simulink model "W06_8_ned"  (R2024b)
settings: Solver=ode4  StartTime=0  StopTime=120  FixedStep=h  RelTol=1e-3
InitFcn:
  | addpath(fullfile(fileparts(fileparts(fileparts(get_param(bdroot, 'FileName')))), '_tools'), fileparts(get_param(bdroot, 'FileName'))); run_alone('W06', bdroot);
StopFcn:
  | W06_plot;
values from neighbouring files (symbols this model uses):
  animate = 1    [W06_0_setup.m]    (also in W06_1_point_run.m = 0; W06_2_sway_run.m = 0; W06_3_thrust_run.m = 0; W06_4_stop_run.m = 0)
  beta_c = pi/2    (= 1.57079632679)    [W06_0_setup.m]    (also in W06_4_stop_run.m = V.beta_c)
  Binv = inv(B)    [W06_0_setup.m]
  bow = [l_f, k_bow, n_bow_max]    [W06_0_setup.m]
  h = 0.02    [W06_0_setup.m]
  k_bow = cfg.k_bow    [W06_0_setup.m]
  k_neg = cfg.k_neg    [W06_0_setup.m]
  k_pos = cfg.k_pos    [W06_0_setup.m]
  Kb = 1    [W06_0_setup.m]
  Kd = 100    [W06_0_setup.m]
  Ki_ned = 120    [W06_0_setup.m]
  Kp = 300    [W06_0_setup.m]
  Kp_ned = 150    [W06_0_setup.m]
  Kp_pos = 0.30    (= 0.3)    [W06_0_setup.m]    (also in W06_4_stop_run.m = V.Kp_pos)
  mp = 25    [W06_0_setup.m]
  n_bow_max = cfg.n_bow_max    [W06_0_setup.m]    (also in W06_1_point_run.m = V.n_bow_max)
  n_max = cfg.n_max    [W06_0_setup.m]
  N_max = 2*y_pont*min(T_max, -T_min)    [W06_0_setup.m]
  n_min = cfg.n_min    [W06_0_setup.m]
  psi_d_cmd = 0    [W06_0_setup.m]    (also in W06_1_point_run.m; W06_8_ned_run.m)
  rp = [0.05 0 -0.35]'    [W06_0_setup.m]
  V_c = 0    [W06_0_setup.m]    (also in W06_4_stop_run.m = V.V_c)
  x0 = zeros(12,1)    [W06_0_setup.m]
  X_max = 120    [W06_0_setup.m]    (also in W06_plot.m = base_var('X_max', 120))
settings Model: Creator=admin  LastModifiedBy=admin
settings DataIOCC: ReturnWorkspaceOutputs=off

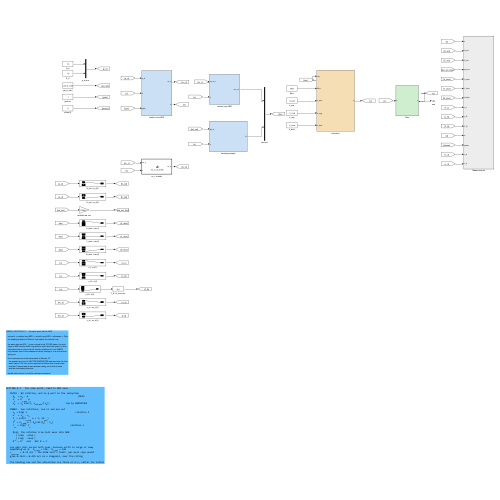
[thumbnail: Simulink's stored preview of the top-level diagram]
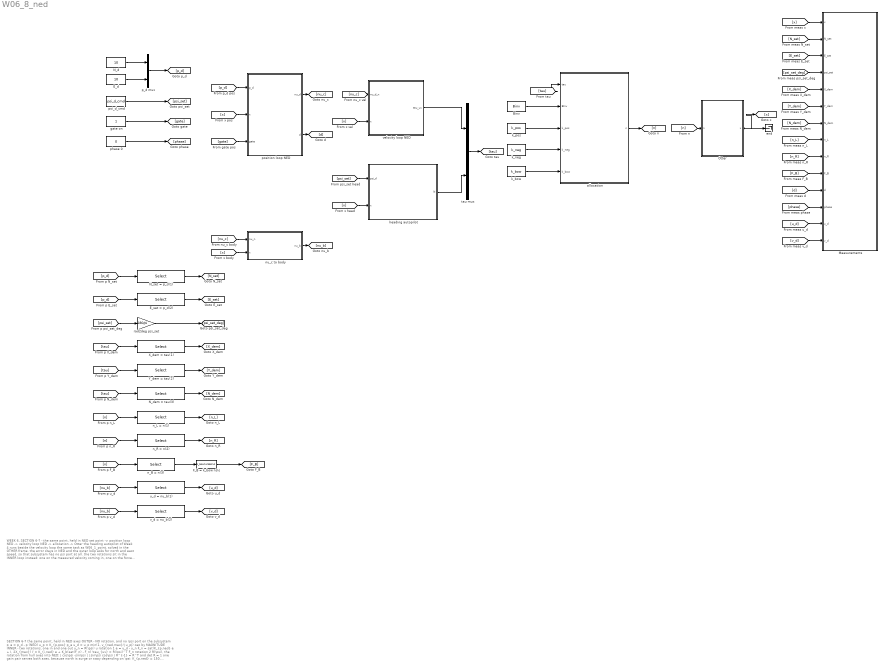
== system W06_8_ned ==
  note: WEEK 6, SECTION 6-7  -  the same point, held in NED
      |
      |    set point -> position loop NED -> velocity loop NED -> allocation -> Otter
      |    the heading autopilot of Week 4 runs beside the velocity loop
      |
      |    the same task as W06_1_point, solved in the OTHER frame. the error
      |    stays in NED and the outer loop asks for north and east speed, so that
      |    subsystem has no psi port at all. the two rotations sit in the INNER
      |    loop instead: one on the measured velocity coming in, one on the force
      |    going out
      |
      |    two consequences, both measurable in Section 6-7:
      |      the speed cap is on the VECTOR MAGNITUDE and must use the slow
      |      axis's value, 0.35 m/s, so the approach is slower than in body axes;
      |      and the PI cannot see its own actuator rating, so its limit is loose
      |      and the anti-windup bites late
      |
      |    double-click a block to read its code and comments
  note: SECTION 6-7   the same point, held in NED axes
      |
      |    OUTER - NO rotation, and no \psi port on the subsystem
      |      p_e  = p_d - p                                     (NED)
      |      \nu_p  = K_{p,pos} p_e
      |      \nu_d  = \nu_p min(1, v_{ned,max}/|\nu_p|)            cap by MAGNITUDE
      |
      |    INNER - two rotations, one in and one out
      |      \nu_n = R(\psi) \nu                                    rotation 1
      |      e   = \nu_d - \nu_n
      |      F_n = sat(K_{p,ned} e + I, 2X_{max})
      |      I' = K_{i,ned} e + K_b(sat(F_n) - F_n)
      |      \tau_{uv} = R(\psi)^T F_n                              rotation 2
      |
      |      R(\psi), the rotation from hull axes into NED:
      |        | cos\psi  -sin\psi |
      |        | sin\psi   cos\psi |
      |      R^{-1} = R^T   and   det R = 1
      |
      |    one gain pair serves both axes, because north is surge or sway
      |    depending on \psi:  K_{p,ned} = 150,  K_{i,ned} = 120
      |    v_{ned,max} = 0.35 m/s - the SLOW axis's limit. per-axis caps would
      |    give 0.35\surd2 = 0.495 m/s on a diagonal, over the rating
      |
      |    the heading law and the allocation are those of 6-3, letter for letter
  Binv : Constant  Value=Binv
  E_d : Constant  Value=10
  E_set = p_d(2) : Selector  InputPortWidth=2  IndexOptions=Index vector (dialog)  Indices=2  OutputSizes=1
  F_B = k_bow n|n| : Fcn  Expr=k_bow*u*abs(u)
  Measurements : Subsystem
  N_d : Constant  Value=10
  N_dem = tau(3) : Selector  InputPortWidth=3  IndexOptions=Index vector (dialog)  Indices=3  OutputSizes=1
  N_set = p_d(1) : Selector  InputPortWidth=2  IndexOptions=Index vector (dialog)  Indices=1  OutputSizes=1
  Otter : Subsystem
  X_dem = tau(1) : Selector  InputPortWidth=3  IndexOptions=Index vector (dialog)  Indices=1  OutputSizes=1
  Y_dem = tau(2) : Selector  InputPortWidth=3  IndexOptions=Index vector (dialog)  Indices=2  OutputSizes=1
  allocation : Subsystem
  end : Terminator
  gate on : Constant
  heading autopilot : Subsystem
  k_bow : Constant  Value=k_bow
  k_neg : Constant  Value=k_neg
  k_pos : Constant  Value=k_pos
  n_B = n(3) : Selector  InputPortWidth=3  IndexOptions=Index vector (dialog)  Indices=3  OutputSizes=1
  n_L = n(1) : Selector  InputPortWidth=3  IndexOptions=Index vector (dialog)  Indices=1  OutputSizes=1
  n_R = n(2) : Selector  InputPortWidth=3  IndexOptions=Index vector (dialog)  Indices=2  OutputSizes=1
  nu_c to body : MATLAB Function  TreatAsAtomicUnit=on
  p_d mux : Mux  Inputs=2
  phase 0 : Constant  Value=0
  position loop NED : Subsystem
  psi_d_cmd : Constant  Value=psi_d_cmd
  rad2deg psi_set : Gain  Gain=180/pi
  tau mux : Mux  Inputs=2
  u_d = nu_b(1) : Selector  InputPortWidth=2  IndexOptions=Index vector (dialog)  Indices=1  OutputSizes=1
  v_d = nu_b(2) : Selector  InputPortWidth=2  IndexOptions=Index vector (dialog)  Indices=2  OutputSizes=1
  velocity loop NED : Subsystem
  wires:
  N_d/1 -> p_d mux/1
  E_d/1 -> p_d mux/2
  p_d mux/1 -> [p_d]
  psi_d_cmd/1 -> [psi_set]
  gate on/1 -> [gate]
  phase 0/1 -> [phase]
  [p_d] -> position loop NED/1(p_d)
  [x] -> position loop NED/2(x)
  [gate] -> position loop NED/3(gate)
  position loop NED/2(d) -> [d]
  position loop NED/1(nu_d) -> [nu_c]
  [nu_c] -> velocity loop NED/1(nu_d_n)
  [x] -> velocity loop NED/2(x)
  [nu_c] -> nu_c to body/1(nu_n)
  [x] -> nu_c to body/2(x)
  nu_c to body/1(nu_b) -> [nu_b]
  [psi_set] -> heading autopilot/1(psi_d)
  [x] -> heading autopilot/2(x)
  velocity loop NED/1(tau_uv) -> tau mux/1
  heading autopilot/1(N) -> tau mux/2
  tau mux/1 -> [tau]
  [tau] -> allocation/1(tau)
  Binv/1 -> allocation/2(Binv)
  k_pos/1 -> allocation/3(k_pos)
  k_neg/1 -> allocation/4(k_neg)
  k_bow/1 -> allocation/5(k_bow)
  allocation/1(n) -> [n]
  [n] -> Otter/1(n)
  Otter/1(x) -> [x], end/1
  [x] -> Measurements/1(x)
  [N_set] -> Measurements/2(N_set)
  [E_set] -> Measurements/3(E_set)
  [psi_set_deg] -> Measurements/4(psi_set)
  [X_dem] -> Measurements/5(X_dem)
  [Y_dem] -> Measurements/6(Y_dem)
  [N_dem] -> Measurements/7(N_dem)
  [n_L] -> Measurements/8(n_L)
  [n_R] -> Measurements/9(n_R)
  [F_B] -> Measurements/10(F_B)
  [d] -> Measurements/11(d)
  [phase] -> Measurements/12(phase)
  [u_d] -> Measurements/13(u_d)
  [v_d] -> Measurements/14(v_d)
  [p_d] -> N_set = p_d(1)/1
  N_set = p_d(1)/1 -> [N_set]
  [p_d] -> E_set = p_d(2)/1
  E_set = p_d(2)/1 -> [E_set]
  [psi_set] -> rad2deg psi_set/1
  rad2deg psi_set/1 -> [psi_set_deg]
  [tau] -> X_dem = tau(1)/1
  X_dem = tau(1)/1 -> [X_dem]
  [tau] -> Y_dem = tau(2)/1
  Y_dem = tau(2)/1 -> [Y_dem]
  [tau] -> N_dem = tau(3)/1
  N_dem = tau(3)/1 -> [N_dem]
  [n] -> n_L = n(1)/1
  n_L = n(1)/1 -> [n_L]
  [n] -> n_R = n(2)/1
  n_R = n(2)/1 -> [n_R]
  [n] -> n_B = n(3)/1
  n_B = n(3)/1 -> F_B = k_bow n|n|/1
  F_B = k_bow n|n|/1 -> [F_B]
  [nu_b] -> u_d = nu_b(1)/1
  u_d = nu_b(1)/1 -> [u_d]
  [nu_b] -> v_d = nu_b(2)/1
  v_d = nu_b(2)/1 -> [v_d]

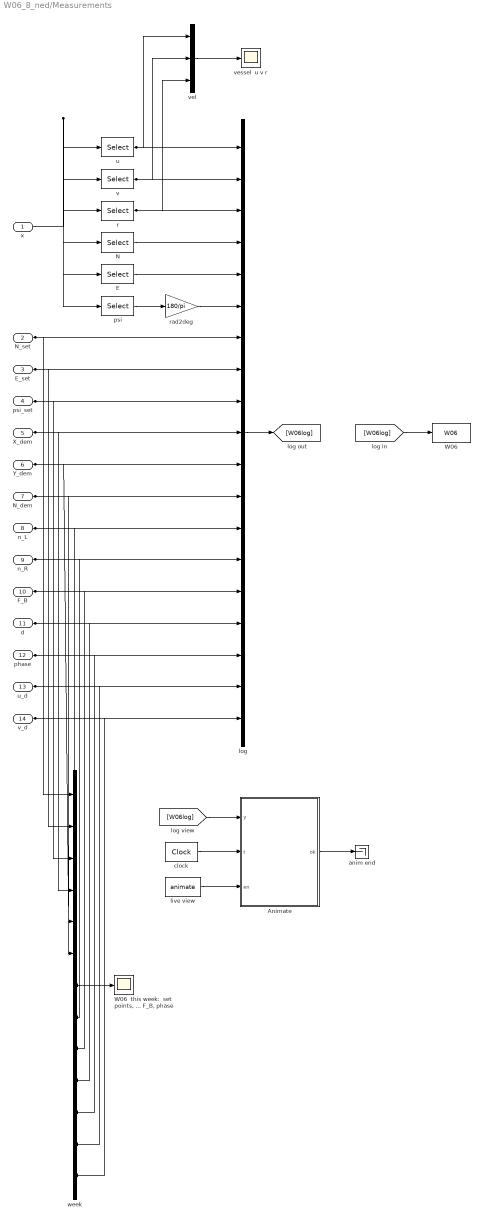
== system W06_8_ned/Measurements ==
  x : Inport
  N_set : Inport  Port=2
  E_set : Inport  Port=3
  psi_set : Inport  Port=4
  X_dem : Inport  Port=5
  Y_dem : Inport  Port=6
  N_dem : Inport  Port=7
  n_L : Inport  Port=8
  n_R : Inport  Port=9
  F_B : Inport  Port=10
  d : Inport  Port=11
  phase : Inport  Port=12
  u_d : Inport  Port=13
  v_d : Inport  Port=14
  Animate : MATLAB Function  TreatAsAtomicUnit=on
  E : Selector  InputPortWidth=12  IndexOptions=Index vector (dialog)  Indices=8  OutputSizes=1
  N : Selector  InputPortWidth=12  IndexOptions=Index vector (dialog)  Indices=7  OutputSizes=1
  W06 : ToWorkspace  VariableName=W06  SaveFormat=Structure With Time  SampleTime=-1
  "W06  this week:  set points, demands, n_L n_R, F_B, phase" : Scope
  anim end : Terminator
  clock : DigitalClock  SampleTime=h
  live view : Constant  Value=animate
  log : Mux  Inputs=19
  psi : Selector  InputPortWidth=12  IndexOptions=Index vector (dialog)  Indices=12  OutputSizes=1
  r : Selector  InputPortWidth=12  IndexOptions=Index vector (dialog)  Indices=6  OutputSizes=1
  rad2deg : Gain  Gain=180/pi
  u : Selector  InputPortWidth=12  IndexOptions=Index vector (dialog)  Indices=1  OutputSizes=1
  v : Selector  InputPortWidth=12  IndexOptions=Index vector (dialog)  Indices=2  OutputSizes=1
  vel : Mux  Inputs=3
  vessel  u v r : Scope
  week : Mux  Inputs=13
  wires:
  x/1 -> u/1, v/1, r/1, N/1, E/1, psi/1
  log/1 -> [W06log]
  [W06log] -> W06/1
  psi/1 -> rad2deg/1
  u/1 -> log/1, vel/1
  v/1 -> log/2, vel/2
  r/1 -> log/3, vel/3
  N/1 -> log/4
  E/1 -> log/5
  rad2deg/1 -> log/6
  N_set/1 -> log/7, week/1
  E_set/1 -> log/8, week/2
  psi_set/1 -> log/9, week/3
  X_dem/1 -> log/10, week/4
  Y_dem/1 -> log/11, week/5
  N_dem/1 -> log/12, week/6
  n_L/1 -> log/13, week/7
  n_R/1 -> log/14, week/8
  F_B/1 -> log/15, week/9
  d/1 -> log/16, week/10
  phase/1 -> log/17, week/11
  u_d/1 -> log/18, week/12
  v_d/1 -> log/19, week/13
  vel/1 -> vessel  u v r/1
  week/1 -> "W06  this week:  set points, demands, n_L n_R, F_B, phase"/1
  [W06log] -> Animate/1(y)
  clock/1 -> Animate/2(t)
  live view/1 -> Animate/3(en)
  Animate/1(ok) -> anim end/1

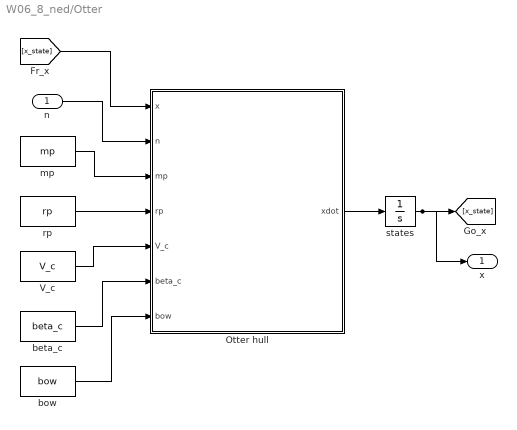
== system W06_8_ned/Otter ==
  n : Inport
  Otter hull : MATLAB Function  TreatAsAtomicUnit=on
  V_c : Constant  Value=V_c
  beta_c : Constant  Value=beta_c
  bow : Constant  Value=bow
  mp : Constant  Value=mp
  rp : Constant  Value=rp
  states : Integrator  InitialCondition=x0
  x : Outport
  wires:
  n/1 -> Otter hull/2(n)
  [x_state] -> Otter hull/1(x)
  bow/1 -> Otter hull/7(bow)
  V_c/1 -> Otter hull/5(V_c)
  mp/1 -> Otter hull/3(mp)
  rp/1 -> Otter hull/4(rp)
  beta_c/1 -> Otter hull/6(beta_c)
  Otter hull/1(xdot) -> states/1
  states/1 -> x/1, [x_state]

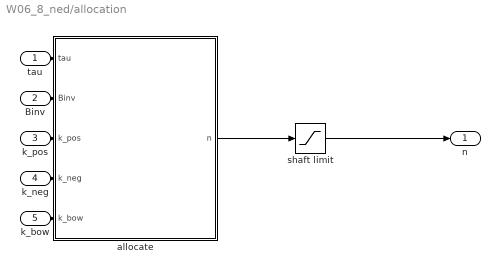
== system W06_8_ned/allocation ==
  tau : Inport
  Binv : Inport  Port=2
  k_pos : Inport  Port=3
  k_neg : Inport  Port=4
  k_bow : Inport  Port=5
  allocate : MATLAB Function  TreatAsAtomicUnit=on
  shaft limit : Saturate  UpperLimit="[ n_max;  n_max;  n_bow_max]"  LowerLimit="[ n_min;  n_min; -n_bow_max]"
  n : Outport
  wires:
  tau/1 -> allocate/1(tau)
  Binv/1 -> allocate/2(Binv)
  k_pos/1 -> allocate/3(k_pos)
  k_neg/1 -> allocate/4(k_neg)
  k_bow/1 -> allocate/5(k_bow)
  allocate/1(n) -> shaft limit/1
  shaft limit/1 -> n/1

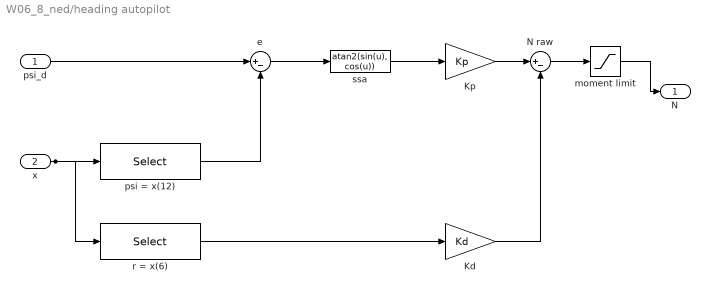
== system W06_8_ned/heading autopilot ==
  psi_d : Inport
  x : Inport  Port=2
  Kd : Gain  Gain=Kd
  Kp : Gain  Gain=Kp
  N raw : Sum  Inputs=|+-
  e : Sum  Inputs=|+-
  moment limit : Saturate  UpperLimit=N_max  LowerLimit=-N_max
  psi = x(12) : Selector  InputPortWidth=12  IndexOptions=Index vector (dialog)  Indices=12  OutputSizes=1
  r = x(6) : Selector  InputPortWidth=12  IndexOptions=Index vector (dialog)  Indices=6  OutputSizes=1
  ssa : Fcn  Expr=atan2(sin(u), cos(u))
  N : Outport
  wires:
  x/1 -> psi = x(12)/1, r = x(6)/1
  psi_d/1 -> e/1
  psi = x(12)/1 -> e/2
  e/1 -> ssa/1
  ssa/1 -> Kp/1
  r = x(6)/1 -> Kd/1
  Kp/1 -> N raw/1
  Kd/1 -> N raw/2
  N raw/1 -> moment limit/1
  moment limit/1 -> N/1

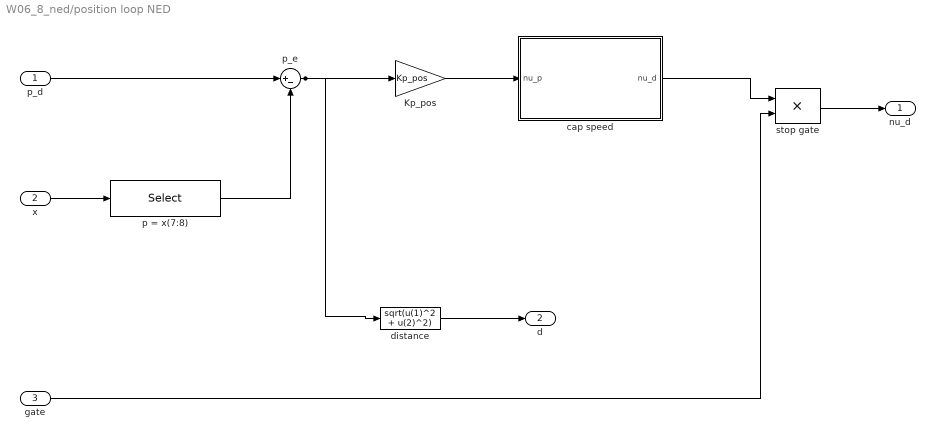
== system W06_8_ned/position loop NED ==
  p_d : Inport
  x : Inport  Port=2
  gate : Inport  Port=3
  Kp_pos : Gain  Gain=Kp_pos
  cap speed : MATLAB Function  TreatAsAtomicUnit=on
  distance : Fcn  Expr=sqrt(u(1)^2 + u(2)^2)
  p = x(7:8) : Selector  InputPortWidth=12  IndexOptions=Index vector (dialog)  Indices=[7 8]  OutputSizes=1
  p_e : Sum  Inputs=|+-
  stop gate : Product
  nu_d : Outport
  d : Outport  Port=2
  wires:
  x/1 -> p = x(7:8)/1
  p_d/1 -> p_e/1
  p = x(7:8)/1 -> p_e/2
  p_e/1 -> Kp_pos/1, distance/1
  Kp_pos/1 -> cap speed/1(nu_p)
  cap speed/1(nu_d) -> stop gate/1
  gate/1 -> stop gate/2
  stop gate/1 -> nu_d/1
  distance/1 -> d/1

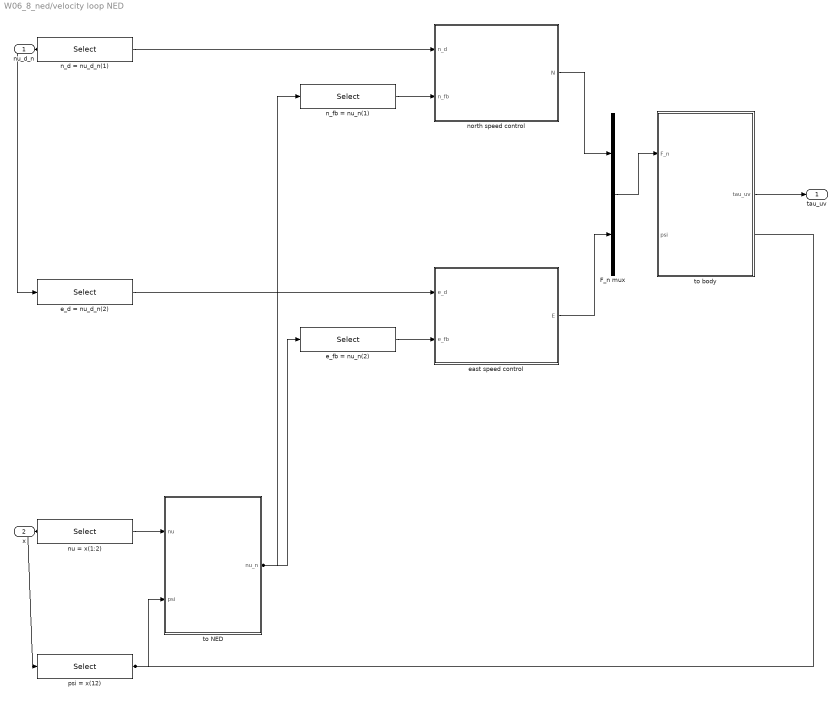
== system W06_8_ned/velocity loop NED ==
  nu_d_n : Inport
  x : Inport  Port=2
  F_n mux : Mux  Inputs=2
  e_d = nu_d_n(2) : Selector  InputPortWidth=2  IndexOptions=Index vector (dialog)  Indices=2  OutputSizes=1
  e_fb = nu_n(2) : Selector  InputPortWidth=2  IndexOptions=Index vector (dialog)  Indices=2  OutputSizes=1
  east speed control : Subsystem
  n_d = nu_d_n(1) : Selector  InputPortWidth=2  IndexOptions=Index vector (dialog)  Indices=1  OutputSizes=1
  n_fb = nu_n(1) : Selector  InputPortWidth=2  IndexOptions=Index vector (dialog)  Indices=1  OutputSizes=1
  north speed control : Subsystem
  nu = x(1:2) : Selector  InputPortWidth=12  IndexOptions=Index vector (dialog)  Indices=[1 2]  OutputSizes=1
  psi = x(12) : Selector  InputPortWidth=12  IndexOptions=Index vector (dialog)  Indices=12  OutputSizes=1
  to NED : MATLAB Function  TreatAsAtomicUnit=on
  to body : MATLAB Function  TreatAsAtomicUnit=on
  tau_uv : Outport
  wires:
  nu_d_n/1 -> n_d = nu_d_n(1)/1, e_d = nu_d_n(2)/1
  x/1 -> nu = x(1:2)/1, psi = x(12)/1
  nu = x(1:2)/1 -> to NED/1(nu)
  psi = x(12)/1 -> to NED/2(psi), to body/2(psi)
  to NED/1(nu_n) -> n_fb = nu_n(1)/1, e_fb = nu_n(2)/1
  n_d = nu_d_n(1)/1 -> north speed control/1(n_d)
  n_fb = nu_n(1)/1 -> north speed control/2(n_fb)
  e_d = nu_d_n(2)/1 -> east speed control/1(e_d)
  e_fb = nu_n(2)/1 -> east speed control/2(e_fb)
  north speed control/1(N) -> F_n mux/1
  east speed control/1(E) -> F_n mux/2
  F_n mux/1 -> to body/1(F_n)
  to body/1(tau_uv) -> tau_uv/1

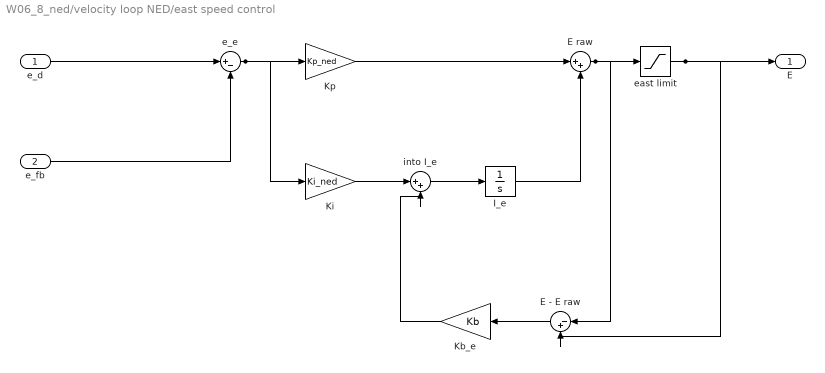
== system W06_8_ned/velocity loop NED/east speed control ==
  e_d : Inport
  e_fb : Inport  Port=2
  E - E raw : Sum  Inputs=|-+
  E raw : Sum  Inputs=|++
  I_e : Integrator
  Kb_e : Gain  Gain=Kb
  Ki : Gain  Gain=Ki_ned
  Kp : Gain  Gain=Kp_ned
  e_e : Sum  Inputs=|+-
  east limit : Saturate  UpperLimit=2*X_max  LowerLimit=-2*X_max
  into I_e : Sum  Inputs=|++
  E : Outport
  wires:
  e_d/1 -> e_e/1
  e_fb/1 -> e_e/2
  e_e/1 -> Kp/1, Ki/1
  Ki/1 -> into I_e/1
  into I_e/1 -> I_e/1
  Kp/1 -> E raw/1
  I_e/1 -> E raw/2
  E raw/1 -> east limit/1, E - E raw/1
  east limit/1 -> E - E raw/2, E/1
  E - E raw/1 -> Kb_e/1
  Kb_e/1 -> into I_e/2

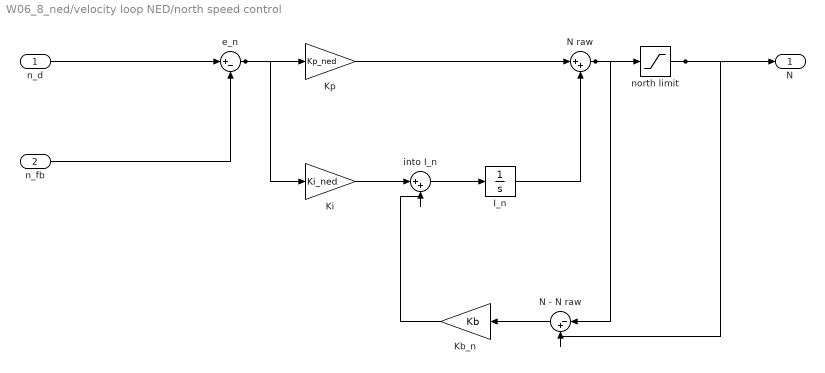
== system W06_8_ned/velocity loop NED/north speed control ==
  n_d : Inport
  n_fb : Inport  Port=2
  I_n : Integrator
  Kb_n : Gain  Gain=Kb
  Ki : Gain  Gain=Ki_ned
  Kp : Gain  Gain=Kp_ned
  N - N raw : Sum  Inputs=|-+
  N raw : Sum  Inputs=|++
  e_n : Sum  Inputs=|+-
  into I_n : Sum  Inputs=|++
  north limit : Saturate  UpperLimit=2*X_max  LowerLimit=-2*X_max
  N : Outport
  wires:
  n_d/1 -> e_n/1
  n_fb/1 -> e_n/2
  e_n/1 -> Kp/1, Ki/1
  Ki/1 -> into I_n/1
  into I_n/1 -> I_n/1
  Kp/1 -> N raw/1
  I_n/1 -> N raw/2
  N raw/1 -> north limit/1, N - N raw/1
  north limit/1 -> N - N raw/2, N/1
  N - N raw/1 -> Kb_n/1
  Kb_n/1 -> into I_n/2

== matlab function W06_8_ned/velocity loop NED/to NED ==
  data: nu input; nu_n output double size=[2 1]; psi input
function nu_n = to_ned(nu, psi)
c = cos(psi);
s = sin(psi);
nu_n = [ c*nu(1) - s*nu(2) ;      % 북쪽으로 가는 빠르기 / speed to the north
         s*nu(1) + c*nu(2) ];     % 동쪽으로 가는 빠르기 / speed to the east
end

== matlab function W06_8_ned/position loop NED/cap speed ==
  data: nu_p input; nu_d output double size=[2 1]; v_ned_max parameter
function nu_d = cap_speed(nu_p, v_ned_max)
%  방향은 그대로, 빠르기만 줄인다 / keep the direction, shrink the speed
sp = sqrt(nu_p(1)^2 + nu_p(2)^2);
if sp > v_ned_max
    nu_d = nu_p * (v_ned_max/sp);
else
    nu_d = nu_p;
end
end

== matlab function W06_8_ned/velocity loop NED/to body ==
  data: F_n input; tau_uv output double size=[2 1]; psi input
function tau_uv = to_body(F_n, psi)
c = cos(psi);
s = sin(psi);
tau_uv = [  c*F_n(1) + s*F_n(2) ;    % 전진 방향의 힘 / along the bow
           -s*F_n(1) + c*F_n(2) ];   % 우현 방향의 힘 / to starboard
end

== matlab function W06_8_ned/nu_c to body ==
  data: nu_n input; nu_b output double size=[2 1]; x input
function nu_b = nu_c_to_body(nu_n, x)
%#codegen
%  같은 속도 명령을 몸체 축에서 읽는다 / the same command, in body axes
%     nu_b = R(psi)' * nu_n,      R(psi) = [c -s; s c]
%  기록 전용이다. 7 절의 제어는 NED 성분을 그대로 쓰고, 회전은 속도
%  고리 **안**에서 두 번 일어난다 / for the log only
psi  = x(6);
c    = cos(psi);   s = sin(psi);
nu_b = [ c  s; -s  c] * nu_n(1:2);
end

== matlab function W06_8_ned/allocation/allocate ==
  data: tau input; n output double size=[3 1]; Binv input; k_pos input; k_neg input; k_bow input
function n = allocate(tau, Binv, k_pos, k_neg, k_bow)
% Run the actuator model backwards: tau -> f -> u -> n.
%
%   forward    u_i = n_i|n_i|      f = K u        tau = B f
%   inverse    f = B^-1 tau        u = K^-1 f     n_i = sign(u_i) sqrt(|u_i|)
%
%   B    = [    1         1       0  ]    f   = [T_L; T_R; F_B]  [N]
%          [    0         0       1  ]    tau = [X; Y; N]        [N, N, N m]
%          [ y_pont   -y_pont   l_f ]
%
% B is square and non-singular (det B = 0.79), so the solution is unique and
% there is no null space to choose within. Binv comes from the setup script,
% which inverts the B that otter_B() derives from the column rule.
f = Binv * tau;

% K is diagonal, so K^-1 is three divisions. Which coefficient applies depends
% on the sign for a stern propeller, because a propeller pushing astern is
% less efficient than the same propeller pushing ahead. It does not depend on
% the sign for the bow unit: a tunnel thruster is symmetric.
k = [k_pos; k_pos; k_bow];
if f(1) < 0, k(1) = k_neg; end
if f(2) < 0, k(2) = k_neg; end

u = f ./ k;

% n_i = sign(u_i) sqrt(|u_i|). The absolute value is not decoration: slide 133
% writes sqrt(u_i), and without the |.| every astern command returns a complex
% shaft speed.
n = sign(u) .* sqrt(abs(u));
end

== matlab function W06_8_ned/Otter/Otter hull ==
  data: x input; xdot output double size=[12 1]; n input; mp input; rp input; V_c input; beta_c input; bow input
function xdot = otter_hull(x, n, mp, rp, V_c, beta_c, bow)
% otter_bow.m: Fossen's otter.m with a bow tunnel thruster added, called
% unchanged from _tools. Three shaft speeds in, tau built inside.
%
%   x     12 states, fed back from the integrator
%   n     shaft speeds [rad/s]: port stern, starboard stern, bow
%   bow   [l3 k3 n3_max], the bow unit's arm, coefficient and speed limit
%
% The sway force and its moment are now rows 2 and 6 of the tau that the
% motion model builds for itself. Nothing is added after the call.
%
% otter_bow.m is not written for code generation, so the call is extrinsic
% and xdot has to be pre-sized for Simulink to know the output width.
coder.extrinsic('otter_bow');

xdot = zeros(12,1);
xdot = otter_bow(x, n, mp, rp, V_c, beta_c, bow);
end

== matlab function W06_8_ned/Measurements/Animate ==
  data: y input; ok output; t input; en input
function ok = Animate(y, t, en)
%#codegen
% Live view of the vessel while the model runs.
%
% A MATLAB Function block cannot plot, so the drawing function is declared
% extrinsic: Simulink calls plain MATLAB rather than generating code for it.
% Set animate = 0 in the setup script to switch the live view off.
%
% y is the whole log vector, in the column order this subsystem builds:
% [u v r N E psi] first, psi in DEGREES, then the week's own signals.
% The wrapper names the columns; nothing else counts them.
coder.extrinsic('W06_animate');
ok = 1;
if en > 0.5
    W06_animate(y, t);
end
end
